simulink library "lib_TerCtrl_MASedp"  (R2026a)
settings: Solver=VariableStepAuto
undefined symbols (not defined in the file): buses_lf, Ps_lf, Qs_lf, vs_lf
libraries: simulink x4, sl_discontinuities x1
settings Model: Creator=atomas  LastModifiedBy=atomas

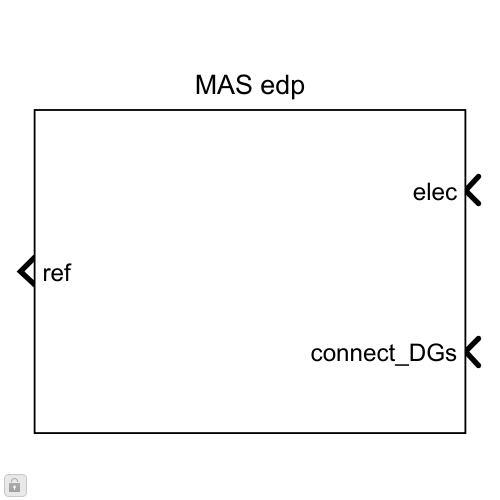
[thumbnail: Simulink's stored preview of the top-level diagram]
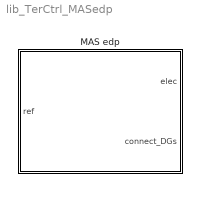
== system lib_TerCtrl_MASedp ==
  MAS edp : Subsystem  VariantControl=MAS edp

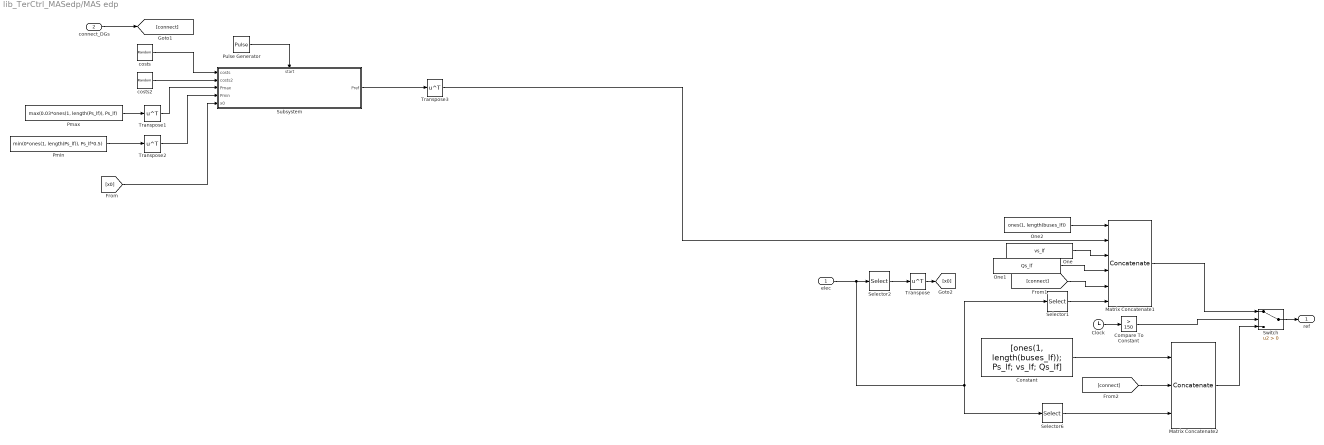
== system lib_TerCtrl_MASedp/MAS edp ==
  elec : Inport
  connect_DGs : Inport  Port=2
  Clock : Clock
  Compare To Constant : simulink/Logic and Bit Operations/Compare To Constant  relop=>  const=150  OutDataTypeStr=boolean
  Constant : Constant  Value=[ones(1, length(buses_lf)); Ps_lf; vs_lf; Qs_lf]  VectorParams1D=off
  Matrix Concatenate1 : Concatenate  NumInputs=6  Mode=Multidimensional array
  Matrix Concatenate2 : Concatenate  NumInputs=3  Mode=Multidimensional array
  One : Constant  Value=vs_lf  VectorParams1D=off  OutDataTypeStr=Inherit: Inherit via back propagation
  One1 : Constant  Value=Qs_lf  VectorParams1D=off  OutDataTypeStr=Inherit: Inherit via back propagation
  One2 : Constant  Value=ones(1, length(buses_lf))  VectorParams1D=off  OutDataTypeStr=Inherit: Inherit via back propagation
  Pmax : Constant  Value=max(0.03*ones(1, length(Ps_lf)), Ps_lf)  VectorParams1D=off
  Pmin : Constant  Value=min(0*ones(1, length(Ps_lf)), Ps_lf*0.5)  VectorParams1D=off
  Pulse Generator : DiscretePulseGenerator  PulseType=Time based  Period=100  PulseWidth=5  PhaseDelay=2
  Selector1 : Selector  NumberOfDimensions=2  InputPortWidth=3  IndexOptions=Index vector (dialog),Select all  Indices=6,1  OutputSizes=1,1
  Selector2 : Selector  NumberOfDimensions=2  InputPortWidth=3  IndexOptions=Index vector (dialog),Select all  Indices=2,1  OutputSizes=1,1
  Selector6 : Selector  NumberOfDimensions=2  InputPortWidth=3  IndexOptions=Index vector (dialog),Select all  Indices=6,1  OutputSizes=1,1
  Subsystem : Subsystem  mask{A=circshift(eye(length(buses_lf)), -1), gainM=0.001}
      settings: PortSchema="{\"entries\":[{\"content\":{\"sides\":[{\"content\":{\"connectorIds\":[\"In1\",\"In2\",\"In3\",\"In4\",\"In5\"]},\"type\":\"ConnectorPlacement.EquallySpacedRectSide\",\"uuid\":\"cdca2cdc-0a32-4006-9eb7-95eef3e074c5\"},{\"content\":{\"connectorIds\":[\"Out1\"],\"side\":\"RIGHT\"},\"type\":\"ConnectorPlacement.EquallySpacedRectSide\",\"uuid\":\"477e4c44-ed13-4581-bb25-eee9ea5698cb\"},{\"content\":{\"connectorIds\":[\"In6\"],\"side\":\"TOP\"},\"type\":\"ConnectorPlacement.EquallySpacedRectSide\",\"uuid\":\"390c7fbe-2640-4698-bec4-03c3001b65dc\"}]},\"type\":\"ConnectorPlacement.EquallySpacedConnector\",\"uuid\":\"648f22ad-3aa2-45b0-803b-7637b6161fb1\"}],\"packageUris\":[\"http://schema.mathworks.com/mf0/Connector/R2020b\"],\"version\":\"1.0\"}"
  Switch : Switch  Criteria=u2 > Threshold  SaturateOnIntegerOverflow=off  InputSameDT=off
  Transpose{,1..3} (4 alike) : Math  Operator=transpose
  costs : UniformRandomNumber  Minimum=0  Seed=(1:length(buses_lf))'  SampleTime=100  VectorParams1D=off
  costs2 : UniformRandomNumber  Minimum=0  Seed=9*(1:length(buses_lf))'  SampleTime=100  VectorParams1D=off
  ref : Outport
  wires:
  Transpose3/1 -> Matrix Concatenate1/2
  Transpose2/1 -> Subsystem/4(Pmin)
  Transpose1/1 -> Subsystem/3(Pmax)
  [x0] -> Subsystem/5(x0)
  Pulse Generator/1 -> Subsystem/6(start)
  Transpose/1 -> [x0]
  Selector2/1 -> Transpose/1
  costs2/1 -> Subsystem/2(costs2)
  costs/1 -> Subsystem/1(costs)
  Subsystem/1(Pref) -> Transpose3/1
  elec/1 -> Selector2/1, Selector1/1, Selector6/1
  connect_DGs/1 -> [connect]
  Matrix Concatenate2/1 -> Switch/3
  Switch/1 -> ref/1
  Constant/1 -> Matrix Concatenate2/1
  Selector6/1 -> Matrix Concatenate2/3
  [connect] -> Matrix Concatenate2/2
  Selector1/1 -> Matrix Concatenate1/6
  [connect] -> Matrix Concatenate1/5
  One2/1 -> Matrix Concatenate1/1
  One1/1 -> Matrix Concatenate1/4
  Pmax/1 -> Transpose1/1
  Pmin/1 -> Transpose2/1
  Matrix Concatenate1/1 -> Switch/1
  One/1 -> Matrix Concatenate1/3
  Compare To Constant/1 -> Switch/2
  Clock/1 -> Compare To Constant/1

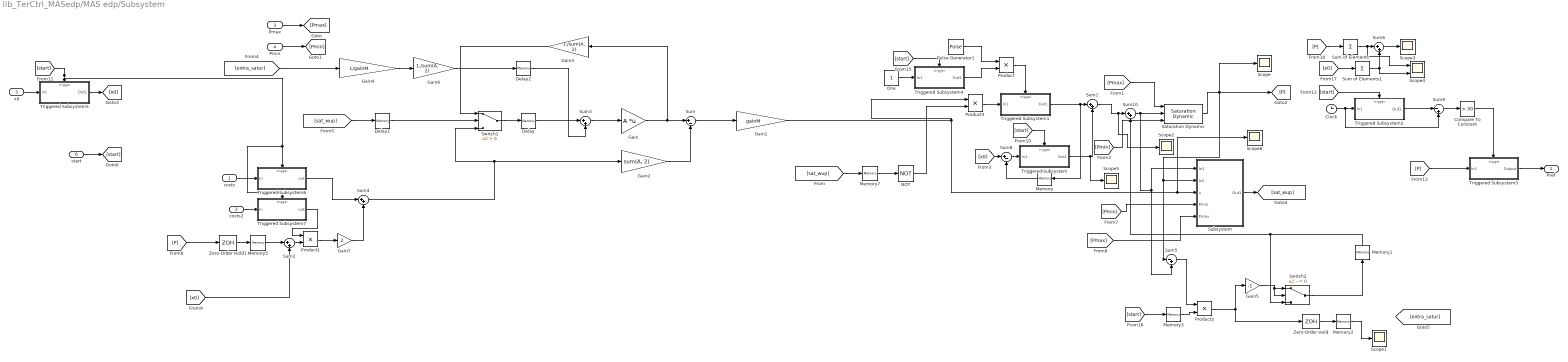
== system lib_TerCtrl_MASedp/MAS edp/Subsystem ==
  costs : Inport
  costs2 : Inport  Port=2
  Pmax : Inport  Port=3
  Pmin : Inport  Port=4
  x0 : Inport  Port=5
  start : Inport  Port=6
  Clock : Clock
  Compare To Constant : simulink/Logic and Bit Operations/Compare To Constant  relop=>  const=30  OutDataTypeStr=boolean
  Delay : Memory
  Delay1 : Memory
  Delay2 : Memory
  Gain : Gain  Gain=A  Multiplication=Matrix(K*u)
  Gain1 : Gain  Gain=gainM
  Gain2 : Gain  Gain=sum(A, 2)
  Gain3 : Gain  Gain=1./sum(A, 2)
  Gain4 : Gain  Gain=1/gainM
  Gain5 : Gain  Gain=-1
  Gain6 : Gain  Gain=1./sum(A, 2)
  Gain7 : Gain  Gain=2
  Memory{,1..3,5,7} (6 alike) : Memory
  NOT : Logic  Operator=NOT  IconShape=distinctive  AllPortsSameDT=off  OutDataTypeStr=boolean
  One : Constant  OutDataTypeStr=Inherit: Inherit via back propagation
  Product{,1..3} (4 alike) : Product
  Pulse Generator1 : DiscretePulseGenerator  PulseType=Time based  Period=0.1  PulseWidth=50
  Saturation Dynamic : sl_discontinuities/Saturation Dynamic  OutMin=[]  OutMax=[]  OutDataTypeStr=Inherit: Same as second input  OutDataType=fixdt(1, 16)  OutScaling=2^-10  DoSatur=off
  Scope{,1..3,5..6} (6 alike) : Scope
      Scope settings: ActiveDisplayYMinimum=-0.00375  ActiveDisplayYMaximum=0.03375
      Scope1 settings: ActiveDisplayYMinimum=-0.00119  ActiveDisplayYMaximum=0.00113
      Scope2 settings: ActiveDisplayYMinimum=-0.00492  ActiveDisplayYMaximum=0.03442  DataLoggingVariableName=ScopeData2
      Scope3 settings: ActiveDisplayYMinimum=-0.01846  ActiveDisplayYMaximum=0.16617  DataLoggingVariableName=ScopeData3
      Scope5 settings: ActiveDisplayYMinimum=-0.01822  ActiveDisplayYMaximum=0.06371
      Scope6 settings: ActiveDisplayYMinimum=-0.00114  ActiveDisplayYMaximum=0.00091  DataLoggingVariableName=ScopeData2
  Scope4 : Scope  NumInputPorts=2
      settings: ActiveDisplayYMinimum=-1  ActiveDisplayYMaximum=1  DataLoggingVariableName=ScopeData4
  Subsystem : Subsystem
  Sum : Sum  Inputs=|+-
  Sum of Elements : Sum  Inputs=+
  Sum of Elements1 : Sum  Inputs=+
  Sum{1..4,6,10} (6 alike) : Sum  Inputs=|++
  Sum5 : Sum  Inputs=|-+
  Sum8 : Sum  Inputs=|+-
  Sum9 : Sum  Inputs=|-+
  Switch1 : Switch  Criteria=u2 > Threshold  SaturateOnIntegerOverflow=off  InputSameDT=off
  Switch2 : Switch  Criteria=u2 ~= 0  SaturateOnIntegerOverflow=off  InputSameDT=off
  Triggered Subsystem : Subsystem  TreatAsAtomicUnit=on
  Triggered Subsystem1 : Subsystem  TreatAsAtomicUnit=on
  Triggered Subsystem2 : Subsystem  TreatAsAtomicUnit=on
  Triggered Subsystem3 : Subsystem  TreatAsAtomicUnit=on
  Triggered Subsystem4 : Subsystem  TreatAsAtomicUnit=on
  Triggered Subsystem5 : Subsystem  TreatAsAtomicUnit=on
  Triggered Subsystem6 : Subsystem  TreatAsAtomicUnit=on
  Triggered Subsystem7 : Subsystem  TreatAsAtomicUnit=on
  Zero-Order Hold : ZeroOrderHold  SampleTime=0.1
  Zero-Order Hold1 : ZeroOrderHold  SampleTime=0.1
  Pref : Outport
  wires:
  Triggered Subsystem7/1(out) -> Product1/1
  costs2/1 -> Triggered Subsystem7/1(in)
  Triggered Subsystem6/1(out) -> Sum4/1
  costs/1 -> Triggered Subsystem6/1(in)
  Gain1/1 -> Subsystem/3(u), Scope6/1, Product3/1
  Sum6/1 -> Scope3/1
  Sum of Elements1/1 -> Sum6/2, Scope4/2
  [P] -> Sum of Elements/1
  [x0] -> Sum of Elements1/1
  Sum of Elements/1 -> Sum6/1, Scope4/1
  Memory3/1 -> Product2/2
  [start] -> Memory3/1
  Sum5/1 -> Product2/1
  Triggered Subsystem5/1(Out1) -> [x0]
  x0/1 -> Triggered Subsystem5/1(x0)
  [start] -> Triggered Subsystem5/Trigger, Triggered Subsystem6/Trigger, Triggered Subsystem7/Trigger
  Product2/1 -> Gain5/1, Zero-Order Hold/1
  Gain5/1 -> Switch2/1, Switch2/2
  Switch2/1 -> Memory1/1
  Memory2/1 -> Scope1/1
  Sum4/1 -> Gain2/1, Switch1/3
  Pulse Generator1/1 -> Product/1
  [start] -> Triggered Subsystem4/Trigger
  One/1 -> Triggered Subsystem4/1(In1)
  Triggered Subsystem4/1(Out1) -> Product/2
  Triggered Subsystem1/1(Out1) -> Sum1/1, Memory/1
  [P] -> Triggered Subsystem3/1(In1)
  Triggered Subsystem3/1(Output) -> Pref/1
  Compare To Constant/1 -> Triggered Subsystem3/Trigger
  Sum9/1 -> Compare To Constant/1
  Triggered Subsystem2/1(Out1) -> Sum9/1
  Clock/1 -> Triggered Subsystem2/1(In1), Sum9/2
  [start] -> Triggered Subsystem2/Trigger
  Sum1/1 -> Sum10/1, Scope2/1
  [start] -> Triggered Subsystem/Trigger
  start/1 -> [start]
  Memory/1 -> Sum8/2
  Sum8/1 -> Triggered Subsystem/1(In1)
  [x0] -> Sum8/1
  Triggered Subsystem/1(Out1) -> Sum1/2, Scope5/1
  Delay/1 -> Sum3/1
  [x0] -> Sum2/2
  Memory5/1 -> Sum2/1
  Sum2/1 -> Product1/2
  [Pmax] -> Subsystem/5(Pmax)
  [Pmin] -> Subsystem/4(Pmin)
  Pmin/1 -> [Pmin]
  Pmax/1 -> [Pmax]
  Product/1 -> Triggered Subsystem1/Trigger
  Sum10/1 -> Subsystem/1(In1), Sum5/2, Saturation Dynamic/2
  Memory1/1 -> Switch2/3, Sum10/2
  NOT/1 -> Product3/2
  Sum/1 -> Gain1/1
  Gain7/1 -> Sum4/2
  Sum3/1 -> Gain/1
  Product3/1 -> Triggered Subsystem1/1(In1)
  [extra_satur] -> Gain4/1
  Product1/1 -> Gain7/1
  Gain4/1 -> Gain6/1
  [Pmax] -> Saturation Dynamic/1
  Memory7/1 -> NOT/1
  Gain6/1 -> Delay2/1
  Subsystem/1(Out1) -> [sat_wup]
  Zero-Order Hold/1 -> Memory2/1
  Delay1/1 -> Switch1/2
  Delay2/1 -> Sum3/2
  Gain2/1 -> Sum/2
  Gain3/1 -> Switch1/1
  [sat_wup] -> Memory7/1
  [P] -> Zero-Order Hold1/1
  Zero-Order Hold1/1 -> Memory5/1
  Saturation Dynamic/1 -> [P], Scope/1, Subsystem/2(In2), Sum5/1
  [Pmin] -> Saturation Dynamic/3
  [sat_wup] -> Delay1/1
  Switch1/1 -> Delay/1
  Gain/1 -> Sum/1, Gain3/1

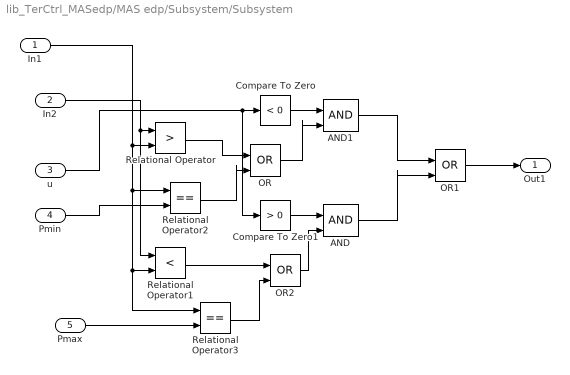
== system lib_TerCtrl_MASedp/MAS edp/Subsystem/Subsystem ==
  In1 : Inport
  In2 : Inport  Port=2
  u : Inport  Port=3
  Pmin : Inport  Port=4
  Pmax : Inport  Port=5
  AND : Logic  IconShape=distinctive  AllPortsSameDT=off  OutDataTypeStr=boolean
  AND1 : Logic  IconShape=distinctive  AllPortsSameDT=off  OutDataTypeStr=boolean
  Compare To Zero : simulink/Logic and Bit Operations/Compare To Zero  relop=<  OutDataTypeStr=boolean
  Compare To Zero1 : simulink/Logic and Bit Operations/Compare To Zero  relop=>  OutDataTypeStr=boolean
  OR : Logic  Operator=OR  IconShape=distinctive  AllPortsSameDT=off  OutDataTypeStr=boolean
  OR1 : Logic  Operator=OR  IconShape=distinctive  AllPortsSameDT=off  OutDataTypeStr=boolean
  OR2 : Logic  Operator=OR  IconShape=distinctive  AllPortsSameDT=off  OutDataTypeStr=boolean
  Relational Operator : RelationalOperator  Operator=>  OutDataTypeStr=boolean  RndMeth=Simplest  InputSameDT=off
  Relational Operator1 : RelationalOperator  Operator=<  OutDataTypeStr=boolean  RndMeth=Simplest  InputSameDT=off
  Relational Operator2 : RelationalOperator  Operator===  OutDataTypeStr=boolean  RndMeth=Simplest  InputSameDT=off
  Relational Operator3 : RelationalOperator  Operator===  OutDataTypeStr=boolean  RndMeth=Simplest  InputSameDT=off
  Out1 : Outport
  wires:
  Pmax/1 -> Relational Operator3/2
  Pmin/1 -> Relational Operator2/2
  Relational Operator2/1 -> OR/2
  AND1/1 -> OR1/1
  AND/1 -> OR1/2
  Relational Operator3/1 -> OR2/2
  Relational Operator1/1 -> OR2/1
  OR2/1 -> AND/2
  OR/1 -> AND1/2
  Relational Operator/1 -> OR/1
  OR1/1 -> Out1/1
  In1/1 -> Relational Operator/2, Relational Operator1/2, Relational Operator3/1, Relational Operator2/1
  Compare To Zero1/1 -> AND/1
  u/1 -> Compare To Zero/1, Compare To Zero1/1
  In2/1 -> Relational Operator/1, Relational Operator1/1
  Compare To Zero/1 -> AND1/1

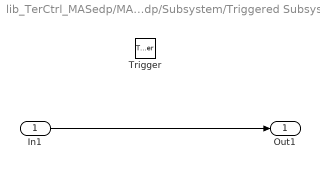
== system lib_TerCtrl_MASedp/MAS edp/Subsystem/Triggered Subsystem ==
  In1 : Inport
  Trigger : TriggerPort  VariantControl=(inherit)
  Out1 : Outport
  wires:
  In1/1 -> Out1/1

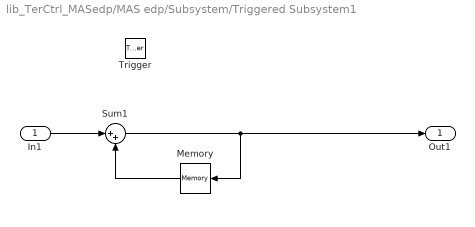
== system lib_TerCtrl_MASedp/MAS edp/Subsystem/Triggered Subsystem1 ==
  In1 : Inport
  Trigger : TriggerPort  VariantControl=(inherit)
  Memory : Memory  InheritSampleTime=on
  Sum1 : Sum  Inputs=|++
  Out1 : Outport
  wires:
  Memory/1 -> Sum1/2
  In1/1 -> Sum1/1
  Sum1/1 -> Memory/1, Out1/1

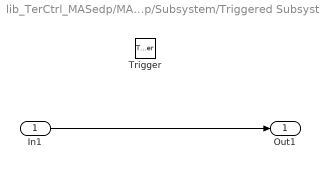
== system lib_TerCtrl_MASedp/MAS edp/Subsystem/Triggered Subsystem2 ==
  In1 : Inport
  Trigger : TriggerPort  VariantControl=(inherit)
  Out1 : Outport
  wires:
  In1/1 -> Out1/1

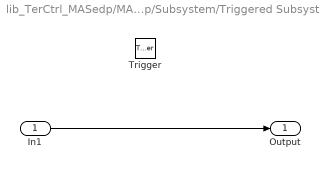
== system lib_TerCtrl_MASedp/MAS edp/Subsystem/Triggered Subsystem3 ==
  In1 : Inport
  Trigger : TriggerPort  VariantControl=(inherit)
  Output : Outport
  wires:
  In1/1 -> Output/1

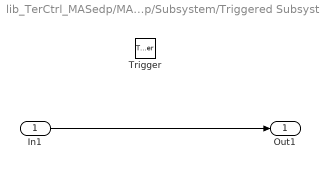
== system lib_TerCtrl_MASedp/MAS edp/Subsystem/Triggered Subsystem4 ==
  In1 : Inport
  Trigger : TriggerPort  VariantControl=(inherit)
  Out1 : Outport
  wires:
  In1/1 -> Out1/1

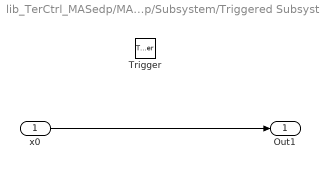
== system lib_TerCtrl_MASedp/MAS edp/Subsystem/Triggered Subsystem5 ==
  x0 : Inport
  Trigger : TriggerPort  VariantControl=(inherit)
  Out1 : Outport
  wires:
  x0/1 -> Out1/1

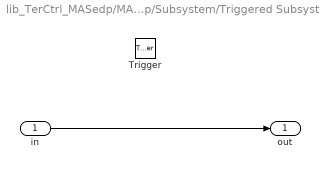
== system lib_TerCtrl_MASedp/MAS edp/Subsystem/Triggered Subsystem6 ==
  in : Inport
  Trigger : TriggerPort  VariantControl=(inherit)
  out : Outport
  wires:
  in/1 -> out/1

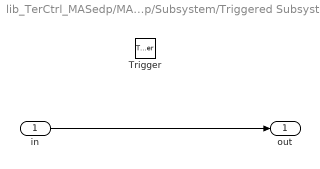
== system lib_TerCtrl_MASedp/MAS edp/Subsystem/Triggered Subsystem7 ==
  in : Inport
  Trigger : TriggerPort  VariantControl=(inherit)
  out : Outport
  wires:
  in/1 -> out/1
